simulink model "quadcopter_ex04_wind_test"  (R2025b)
settings: Solver=ode23t  StartTime=0.0  StopTime=timespot_spl(end)+2  FixedStep=0.01  MaxStep=1e-2  RelTol=1e-3  AbsTol=1e-3
PreLoadFcn:
  | [waypoints, timespot_spl, spline_data, spline_yaw, wayp_path_vis] = quadcopter_package_select_trajectory(2,true);
  | disp('Loaded path 2, round trip');
model workspace (MATLAB code in the model file):
  | load('xy_data_membrane.mat');
values from neighbouring files (symbols this model uses):
  wind_speed = 12    [quadcopter_ex04_wind_test_code.m]
undefined symbols (not defined in the file or in its folder): air_rho, battery_capacity, drone_leg, filtD_altitude, filtD_attitude, filtD_motor, filtD_position, filtD_yaw, filtM_altitude, filtM_attitude, filtM_position, filtM_yaw, filtSpd_motor, kd_altitude, kd_attitude, kd_motor, kd_position, kd_yaw, ki_altitude, ki_attitude, ki_motor, ki_position, ki_yaw, kp_altitude, kp_attitude, kp_motor, kp_position, kp_yaw, limit_altitude, limit_attitude, limit_motor, limit_yaw, pkgDensity, pkgSize, planedepth, pos2attitude, propeller, qc_motor, qd_area, qd_drag, spline_data, spline_yaw, timespot_spl, waypoints, X, Y, Z
libraries: sm_lib x77, nesl_utility x30, fl_lib x13, slpidlib x9, quadcopter_library x6, ee_lib x4, simulink x2, batteryecm_lib x1
(part 4 of 4)

== system quadcopter_ex04_wind_test/Quadcopter/Electrical/Control1 ==
  ref : Inport
  meas : Inport  Port=2
  Add : Sum  Inputs=+-
  Control : slpidlib/PID Controller  Controller=PID  Form=Parallel  TimeDomain=Continuous-time  UseExternalTs=off  SampleTime=-1  IntegratorMethod=Forward Euler  FilterMethod=Forward Euler  ControllerParametersSource=internal  P=kp  I=ki  UseKiTs=off  D=kd  UseExternalDerivativeSource=off  N=f_deriv  UseFilter=on  TunerSelectOption=Transfer Function Based (PID Tuner App)  ZeroCross=off  InitialConditionSource=internal  InitialConditionForIntegrator=0  InitialConditionForFilter=0  DifferentiatorICPrevScaledInput=0  ExternalReset=none  TrackingMode=off  Kt=1  LimitOutput=on  SatLimitsSource=internal  UpperSaturationLimit=max_trq_cmd  LowerSaturationLimit=-max_trq_cmd  LinearizeAsGain=on  AntiWindupMode=clamping  Kb=1  LimitIntegrator=off  UpperIntegratorSaturationLimit=inf  LowerIntegratorSaturationLimit=-inf  POutMin=[]  POutMax=[]  IOutMin=[]  IOutMax=[]  DOutMin=[]  DOutMax=[]  NOutMin=[]  NOutMax=[]  SumOutMin=[]  SumOutMax=[]  SaturationOutMin=[]  SaturationOutMax=[]  PParamMin=[]  PParamMax=[]  IParamMin=[]  IParamMax=[]  DParamMin=[]  DParamMax=[]  NParamMin=[]  NParamMax=[]  KbParamMin=[]  KbParamMax=[]  KtParamMin=[]  KtParamMax=[]  KbOutMin=[]  KbOutMax=[]  KtOutMin=[]  KtOutMax=[]  IntegratorOutMin=[]  IntegratorOutMax=[]  FilterOutMin=[]  FilterOutMax=[]  SumI1OutMin=[]  SumI1OutMax=[]  SumI2OutMin=[]  SumI2OutMax=[]  SumI3OutMin=[]  SumI3OutMax=[]  SumI4OutMin=[]  SumI4OutMax=[]  SumDOutMin=[]  SumDOutMax=[]  DifferentiatorOutMin=[]  DifferentiatorOutMax=[]  FilterDiffOutCoefMin=[]  FilterDiffOutCoefMax=[]  ReciprocalOutMin=[]  ReciprocalOutMax=[]  SumDenOutMin=[]  SumDenOutMax=[]  SumNumOutMin=[]  SumNumOutMax=[]  DivideOutMin=[]  DivideOutMax=[]  UdiffTsProdOutMin=[]  UdiffTsProdOutMax=[]  NTsProdOutMin=[]  NTsProdOutMax=[]  UintegralTsProdOutMin=[]  UintegralTsProdOutMax=[]  UngainTsProdOutMin=[]  UngainTsProdOutMax=[]  ClampingZeroOutDataTypeStr=Inherit: Inherit via back propagation  ClampingZeroOutMin=[]  ClampingZeroOutMax=[]  FilterDenConstantOutDataTypeStr=Inherit: Inherit via back propagation  FilterDenConstantOutMin=[]  FilterDenConstantOutMax=[]  PCopyOutDataTypeStr=Inherit: Inherit via back propagation  PCopyOutMin=[]  PCopyOutMax=[]  NCopyOutDataTypeStr=Inherit: Inherit via back propagation  NCopyOutMin=[]  NCopyOutMax=[]  IntegratorContinuousStateAttributes=''  IntegratorStateMustResolveToSignalObject=off  IntegratorRTWStateStorageClass=Auto  FilterContinuousStateAttributes=''  FilterStateMustResolveToSignalObject=off  FilterRTWStateStorageClass=Auto  ParallelPVariant=InternalParameters  IdealPVariant=Disabled  IVariant=InternalParameters  DVariant=InternalParameters  IntegratorVariant=Continuous  SatVariant=Enabled  AWVariant=ContClampingParallel  PCopyVariant=Disabled  TRVariant=Disabled  FdbkBlocksVariant=Forward  IdealPFdbkVariant=Disabled  SatFdbkVariant=Disabled  DerivativeFilterVariant=ContFilter  NVariant=InternalParameters  NCopyVariant=Disabled  FilterICVariant=InternalICsFilter  IntegratorICVariant=InternalICs  ExternalResetVariant=Disabled  TRSumVariant=Passthrough  SumFdbkVariant=Disabled  SumVariant=Sum_PID  TsampFilterVariant=InternalTs  TsampNgainVariant=Passthrough  TsampIntegralVariant=Disabled_SignalSpec  ExternalSaturationOutDataTypeStr=Inherit: Same as second input  DerivativeSourceVariant=ErrorSignal  PreIntVariant=InternalPreInt
  Mux : Mux  Inputs=2
  Scope : Scope  NumInputPorts=3
      settings: ActiveDisplayYMinimum=-575.93509  ActiveDisplayYMaximum=5183.41577  DataLoggingVariableName=ScopeData3
  Transfer Fcn1 : TransferFcn  Denominator=[f_spd 1]
  torque : Outport
  wires:
  Control/1 -> torque/1, Scope/3  "torque"
  meas/1 -> Transfer Fcn1/1  "Meas"
  ref/1 -> Add/1, Mux/1  "Ref"
  Add/1 -> Scope/2, Control/1  "error"
  Mux/1 -> Scope/1
  Transfer Fcn1/1 -> Add/2, Mux/2

== system quadcopter_ex04_wind_test/Quadcopter/Electrical/Control2 ==
  ref : Inport
  meas : Inport  Port=2
  Add : Sum  Inputs=+-
  Control : slpidlib/PID Controller  Controller=PID  Form=Parallel  TimeDomain=Continuous-time  UseExternalTs=off  SampleTime=-1  IntegratorMethod=Forward Euler  FilterMethod=Forward Euler  ControllerParametersSource=internal  P=kp  I=ki  UseKiTs=off  D=kd  UseExternalDerivativeSource=off  N=f_deriv  UseFilter=on  TunerSelectOption=Transfer Function Based (PID Tuner App)  ZeroCross=off  InitialConditionSource=internal  InitialConditionForIntegrator=0  InitialConditionForFilter=0  DifferentiatorICPrevScaledInput=0  ExternalReset=none  TrackingMode=off  Kt=1  LimitOutput=on  SatLimitsSource=internal  UpperSaturationLimit=max_trq_cmd  LowerSaturationLimit=-max_trq_cmd  LinearizeAsGain=on  AntiWindupMode=clamping  Kb=1  LimitIntegrator=off  UpperIntegratorSaturationLimit=inf  LowerIntegratorSaturationLimit=-inf  POutMin=[]  POutMax=[]  IOutMin=[]  IOutMax=[]  DOutMin=[]  DOutMax=[]  NOutMin=[]  NOutMax=[]  SumOutMin=[]  SumOutMax=[]  SaturationOutMin=[]  SaturationOutMax=[]  PParamMin=[]  PParamMax=[]  IParamMin=[]  IParamMax=[]  DParamMin=[]  DParamMax=[]  NParamMin=[]  NParamMax=[]  KbParamMin=[]  KbParamMax=[]  KtParamMin=[]  KtParamMax=[]  KbOutMin=[]  KbOutMax=[]  KtOutMin=[]  KtOutMax=[]  IntegratorOutMin=[]  IntegratorOutMax=[]  FilterOutMin=[]  FilterOutMax=[]  SumI1OutMin=[]  SumI1OutMax=[]  SumI2OutMin=[]  SumI2OutMax=[]  SumI3OutMin=[]  SumI3OutMax=[]  SumI4OutMin=[]  SumI4OutMax=[]  SumDOutMin=[]  SumDOutMax=[]  DifferentiatorOutMin=[]  DifferentiatorOutMax=[]  FilterDiffOutCoefMin=[]  FilterDiffOutCoefMax=[]  ReciprocalOutMin=[]  ReciprocalOutMax=[]  SumDenOutMin=[]  SumDenOutMax=[]  SumNumOutMin=[]  SumNumOutMax=[]  DivideOutMin=[]  DivideOutMax=[]  UdiffTsProdOutMin=[]  UdiffTsProdOutMax=[]  NTsProdOutMin=[]  NTsProdOutMax=[]  UintegralTsProdOutMin=[]  UintegralTsProdOutMax=[]  UngainTsProdOutMin=[]  UngainTsProdOutMax=[]  ClampingZeroOutDataTypeStr=Inherit: Inherit via back propagation  ClampingZeroOutMin=[]  ClampingZeroOutMax=[]  FilterDenConstantOutDataTypeStr=Inherit: Inherit via back propagation  FilterDenConstantOutMin=[]  FilterDenConstantOutMax=[]  PCopyOutDataTypeStr=Inherit: Inherit via back propagation  PCopyOutMin=[]  PCopyOutMax=[]  NCopyOutDataTypeStr=Inherit: Inherit via back propagation  NCopyOutMin=[]  NCopyOutMax=[]  IntegratorContinuousStateAttributes=''  IntegratorStateMustResolveToSignalObject=off  IntegratorRTWStateStorageClass=Auto  FilterContinuousStateAttributes=''  FilterStateMustResolveToSignalObject=off  FilterRTWStateStorageClass=Auto  ParallelPVariant=InternalParameters  IdealPVariant=Disabled  IVariant=InternalParameters  DVariant=InternalParameters  IntegratorVariant=Continuous  SatVariant=Enabled  AWVariant=ContClampingParallel  PCopyVariant=Disabled  TRVariant=Disabled  FdbkBlocksVariant=Forward  IdealPFdbkVariant=Disabled  SatFdbkVariant=Disabled  DerivativeFilterVariant=ContFilter  NVariant=InternalParameters  NCopyVariant=Disabled  FilterICVariant=InternalICsFilter  IntegratorICVariant=InternalICs  ExternalResetVariant=Disabled  TRSumVariant=Passthrough  SumFdbkVariant=Disabled  SumVariant=Sum_PID  TsampFilterVariant=InternalTs  TsampNgainVariant=Passthrough  TsampIntegralVariant=Disabled_SignalSpec  ExternalSaturationOutDataTypeStr=Inherit: Same as second input  DerivativeSourceVariant=ErrorSignal  PreIntVariant=InternalPreInt
  Mux : Mux  Inputs=2
  Scope : Scope  NumInputPorts=3
      settings: ActiveDisplayYMinimum=-51413.90485  ActiveDisplayYMaximum=107953.94315  DataLoggingVariableName=ScopeData3
  Transfer Fcn1 : TransferFcn  Denominator=[f_spd 1]
  torque : Outport
  wires:
  Control/1 -> torque/1, Scope/3  "torque"
  ref/1 -> Add/1, Mux/1
  Add/1 -> Scope/2, Control/1  "error"
  Mux/1 -> Scope/1
  meas/1 -> Transfer Fcn1/1
  Transfer Fcn1/1 -> Add/2, Mux/2

== system quadcopter_ex04_wind_test/Quadcopter/Electrical/Control3 ==
  ref : Inport
  meas : Inport  Port=2
  Add : Sum  Inputs=+-
  Control : slpidlib/PID Controller  Controller=PID  Form=Parallel  TimeDomain=Continuous-time  UseExternalTs=off  SampleTime=-1  IntegratorMethod=Forward Euler  FilterMethod=Forward Euler  ControllerParametersSource=internal  P=kp  I=ki  UseKiTs=off  D=kd  UseExternalDerivativeSource=off  N=f_deriv  UseFilter=on  TunerSelectOption=Transfer Function Based (PID Tuner App)  ZeroCross=off  InitialConditionSource=internal  InitialConditionForIntegrator=0  InitialConditionForFilter=0  DifferentiatorICPrevScaledInput=0  ExternalReset=none  TrackingMode=off  Kt=1  LimitOutput=on  SatLimitsSource=internal  UpperSaturationLimit=max_trq_cmd  LowerSaturationLimit=-max_trq_cmd  LinearizeAsGain=on  AntiWindupMode=clamping  Kb=1  LimitIntegrator=off  UpperIntegratorSaturationLimit=inf  LowerIntegratorSaturationLimit=-inf  POutMin=[]  POutMax=[]  IOutMin=[]  IOutMax=[]  DOutMin=[]  DOutMax=[]  NOutMin=[]  NOutMax=[]  SumOutMin=[]  SumOutMax=[]  SaturationOutMin=[]  SaturationOutMax=[]  PParamMin=[]  PParamMax=[]  IParamMin=[]  IParamMax=[]  DParamMin=[]  DParamMax=[]  NParamMin=[]  NParamMax=[]  KbParamMin=[]  KbParamMax=[]  KtParamMin=[]  KtParamMax=[]  KbOutMin=[]  KbOutMax=[]  KtOutMin=[]  KtOutMax=[]  IntegratorOutMin=[]  IntegratorOutMax=[]  FilterOutMin=[]  FilterOutMax=[]  SumI1OutMin=[]  SumI1OutMax=[]  SumI2OutMin=[]  SumI2OutMax=[]  SumI3OutMin=[]  SumI3OutMax=[]  SumI4OutMin=[]  SumI4OutMax=[]  SumDOutMin=[]  SumDOutMax=[]  DifferentiatorOutMin=[]  DifferentiatorOutMax=[]  FilterDiffOutCoefMin=[]  FilterDiffOutCoefMax=[]  ReciprocalOutMin=[]  ReciprocalOutMax=[]  SumDenOutMin=[]  SumDenOutMax=[]  SumNumOutMin=[]  SumNumOutMax=[]  DivideOutMin=[]  DivideOutMax=[]  UdiffTsProdOutMin=[]  UdiffTsProdOutMax=[]  NTsProdOutMin=[]  NTsProdOutMax=[]  UintegralTsProdOutMin=[]  UintegralTsProdOutMax=[]  UngainTsProdOutMin=[]  UngainTsProdOutMax=[]  ClampingZeroOutDataTypeStr=Inherit: Inherit via back propagation  ClampingZeroOutMin=[]  ClampingZeroOutMax=[]  FilterDenConstantOutDataTypeStr=Inherit: Inherit via back propagation  FilterDenConstantOutMin=[]  FilterDenConstantOutMax=[]  PCopyOutDataTypeStr=Inherit: Inherit via back propagation  PCopyOutMin=[]  PCopyOutMax=[]  NCopyOutDataTypeStr=Inherit: Inherit via back propagation  NCopyOutMin=[]  NCopyOutMax=[]  IntegratorContinuousStateAttributes=''  IntegratorStateMustResolveToSignalObject=off  IntegratorRTWStateStorageClass=Auto  FilterContinuousStateAttributes=''  FilterStateMustResolveToSignalObject=off  FilterRTWStateStorageClass=Auto  ParallelPVariant=InternalParameters  IdealPVariant=Disabled  IVariant=InternalParameters  DVariant=InternalParameters  IntegratorVariant=Continuous  SatVariant=Enabled  AWVariant=ContClampingParallel  PCopyVariant=Disabled  TRVariant=Disabled  FdbkBlocksVariant=Forward  IdealPFdbkVariant=Disabled  SatFdbkVariant=Disabled  DerivativeFilterVariant=ContFilter  NVariant=InternalParameters  NCopyVariant=Disabled  FilterICVariant=InternalICsFilter  IntegratorICVariant=InternalICs  ExternalResetVariant=Disabled  TRSumVariant=Passthrough  SumFdbkVariant=Disabled  SumVariant=Sum_PID  TsampFilterVariant=InternalTs  TsampNgainVariant=Passthrough  TsampIntegralVariant=Disabled_SignalSpec  ExternalSaturationOutDataTypeStr=Inherit: Same as second input  DerivativeSourceVariant=ErrorSignal  PreIntVariant=InternalPreInt
  Mux : Mux  Inputs=2
  Scope : Scope  NumInputPorts=3
      settings: ActiveDisplayYMinimum=-734.86159  ActiveDisplayYMaximum=6613.7543  DataLoggingVariableName=ScopeData3
  Transfer Fcn1 : TransferFcn  Denominator=[f_spd 1]
  torque : Outport
  wires:
  Control/1 -> torque/1, Scope/3  "torque"
  ref/1 -> Add/1, Mux/1
  Add/1 -> Scope/2, Control/1  "error"
  Mux/1 -> Scope/1
  meas/1 -> Transfer Fcn1/1
  Transfer Fcn1/1 -> Add/2, Mux/2

== system quadcopter_ex04_wind_test/Quadcopter/Electrical/Control4 ==
  ref : Inport
  meas : Inport  Port=2
  Add : Sum  Inputs=+-
  Control : slpidlib/PID Controller  Controller=PID  Form=Parallel  TimeDomain=Continuous-time  UseExternalTs=off  SampleTime=-1  IntegratorMethod=Forward Euler  FilterMethod=Forward Euler  ControllerParametersSource=internal  P=kp  I=ki  UseKiTs=off  D=kd  UseExternalDerivativeSource=off  N=f_deriv  UseFilter=on  TunerSelectOption=Transfer Function Based (PID Tuner App)  ZeroCross=off  InitialConditionSource=internal  InitialConditionForIntegrator=0  InitialConditionForFilter=0  DifferentiatorICPrevScaledInput=0  ExternalReset=none  TrackingMode=off  Kt=1  LimitOutput=on  SatLimitsSource=internal  UpperSaturationLimit=max_trq_cmd  LowerSaturationLimit=-max_trq_cmd  LinearizeAsGain=on  AntiWindupMode=clamping  Kb=1  LimitIntegrator=off  UpperIntegratorSaturationLimit=inf  LowerIntegratorSaturationLimit=-inf  POutMin=[]  POutMax=[]  IOutMin=[]  IOutMax=[]  DOutMin=[]  DOutMax=[]  NOutMin=[]  NOutMax=[]  SumOutMin=[]  SumOutMax=[]  SaturationOutMin=[]  SaturationOutMax=[]  PParamMin=[]  PParamMax=[]  IParamMin=[]  IParamMax=[]  DParamMin=[]  DParamMax=[]  NParamMin=[]  NParamMax=[]  KbParamMin=[]  KbParamMax=[]  KtParamMin=[]  KtParamMax=[]  KbOutMin=[]  KbOutMax=[]  KtOutMin=[]  KtOutMax=[]  IntegratorOutMin=[]  IntegratorOutMax=[]  FilterOutMin=[]  FilterOutMax=[]  SumI1OutMin=[]  SumI1OutMax=[]  SumI2OutMin=[]  SumI2OutMax=[]  SumI3OutMin=[]  SumI3OutMax=[]  SumI4OutMin=[]  SumI4OutMax=[]  SumDOutMin=[]  SumDOutMax=[]  DifferentiatorOutMin=[]  DifferentiatorOutMax=[]  FilterDiffOutCoefMin=[]  FilterDiffOutCoefMax=[]  ReciprocalOutMin=[]  ReciprocalOutMax=[]  SumDenOutMin=[]  SumDenOutMax=[]  SumNumOutMin=[]  SumNumOutMax=[]  DivideOutMin=[]  DivideOutMax=[]  UdiffTsProdOutMin=[]  UdiffTsProdOutMax=[]  NTsProdOutMin=[]  NTsProdOutMax=[]  UintegralTsProdOutMin=[]  UintegralTsProdOutMax=[]  UngainTsProdOutMin=[]  UngainTsProdOutMax=[]  ClampingZeroOutDataTypeStr=Inherit: Inherit via back propagation  ClampingZeroOutMin=[]  ClampingZeroOutMax=[]  FilterDenConstantOutDataTypeStr=Inherit: Inherit via back propagation  FilterDenConstantOutMin=[]  FilterDenConstantOutMax=[]  PCopyOutDataTypeStr=Inherit: Inherit via back propagation  PCopyOutMin=[]  PCopyOutMax=[]  NCopyOutDataTypeStr=Inherit: Inherit via back propagation  NCopyOutMin=[]  NCopyOutMax=[]  IntegratorContinuousStateAttributes=''  IntegratorStateMustResolveToSignalObject=off  IntegratorRTWStateStorageClass=Auto  FilterContinuousStateAttributes=''  FilterStateMustResolveToSignalObject=off  FilterRTWStateStorageClass=Auto  ParallelPVariant=InternalParameters  IdealPVariant=Disabled  IVariant=InternalParameters  DVariant=InternalParameters  IntegratorVariant=Continuous  SatVariant=Enabled  AWVariant=ContClampingParallel  PCopyVariant=Disabled  TRVariant=Disabled  FdbkBlocksVariant=Forward  IdealPFdbkVariant=Disabled  SatFdbkVariant=Disabled  DerivativeFilterVariant=ContFilter  NVariant=InternalParameters  NCopyVariant=Disabled  FilterICVariant=InternalICsFilter  IntegratorICVariant=InternalICs  ExternalResetVariant=Disabled  TRSumVariant=Passthrough  SumFdbkVariant=Disabled  SumVariant=Sum_PID  TsampFilterVariant=InternalTs  TsampNgainVariant=Passthrough  TsampIntegralVariant=Disabled_SignalSpec  ExternalSaturationOutDataTypeStr=Inherit: Same as second input  DerivativeSourceVariant=ErrorSignal  PreIntVariant=InternalPreInt
  Mux : Mux  Inputs=2
  Scope : Scope  NumInputPorts=3
      settings: ActiveDisplayYMinimum=3391.57745  ActiveDisplayYMaximum=7073.87438  DataLoggingVariableName=ScopeData3
  Transfer Fcn1 : TransferFcn  Denominator=[f_spd 1]
  torque : Outport
  wires:
  Control/1 -> torque/1, Scope/3  "torque"
  ref/1 -> Add/1, Mux/1
  Add/1 -> Scope/2, Control/1  "error"
  Mux/1 -> Scope/1
  meas/1 -> Transfer Fcn1/1
  Transfer Fcn1/1 -> Add/2, Mux/2

== system quadcopter_ex04_wind_test/Quadcopter/Electrical/Sensing Temperature ==
  PS-Simulink Converter : nesl_utility/PS-Simulink Converter  PhysicalDomain=network_engine_domain  SubClassName=ps_output  LeftPortType=input  RightPortType=output  PseudoPeriodic=off  Frequencies=[]  VectorFormat=1-D array  Unit=inherit  AffineConversion=off
  Temperature Sensor : fl_lib/Thermal/Thermal Sensors/Temperature Sensor  temperature_measure=foundation.enum.MeasurementReference.difference
  Thermal Reference : fl_lib/Thermal/Thermal Elements/Thermal Reference
  A : PMIOPort  Side=Left
  T : Outport
  wires:
  PS-Simulink Converter/1 -> T/1
  connections:
  Thermal Reference/LConn1 -- Temperature Sensor/RConn1
  Temperature Sensor/RConn2 -- PS-Simulink Converter/LConn1
  A/RConn1 -- Temperature Sensor/LConn1

== system quadcopter_ex04_wind_test/Quadcopter/Electrical/Sensor M1 ==
  Current Sensor : fl_lib/Electrical/Electrical Sensors/Current Sensor
  PS-Simulink Converter3 : nesl_utility/PS-Simulink Converter  PhysicalDomain=network_engine_domain  SubClassName=ps_output  LeftPortType=input  RightPortType=output  PseudoPeriodic=off  Frequencies=[]  VectorFormat=1-D array  Unit=inherit  AffineConversion=off
  + : PMIOPort  Side=Left
  - : PMIOPort  Port=2  Side=Right
  i : Outport
  wires:
  PS-Simulink Converter3/1 -> i/1
  connections:
  +/RConn1 -- Current Sensor/LConn1
  Current Sensor/RConn2 -- -/RConn1
  PS-Simulink Converter3/LConn1 -- Current Sensor/RConn1

== system quadcopter_ex04_wind_test/Quadcopter/Electrical/Sensor M2 ==
  Current Sensor : fl_lib/Electrical/Electrical Sensors/Current Sensor
  PS-Simulink Converter3 : nesl_utility/PS-Simulink Converter  PhysicalDomain=network_engine_domain  SubClassName=ps_output  LeftPortType=input  RightPortType=output  PseudoPeriodic=off  Frequencies=[]  VectorFormat=1-D array  Unit=inherit  AffineConversion=off
  + : PMIOPort  Side=Left
  - : PMIOPort  Port=2  Side=Right
  i : Outport
  wires:
  PS-Simulink Converter3/1 -> i/1
  connections:
  PS-Simulink Converter3/LConn1 -- Current Sensor/RConn1
  Current Sensor/RConn2 -- -/RConn1
  +/RConn1 -- Current Sensor/LConn1

== system quadcopter_ex04_wind_test/Quadcopter/Electrical/Sensor M3 ==
  Current Sensor : fl_lib/Electrical/Electrical Sensors/Current Sensor
  PS-Simulink Converter3 : nesl_utility/PS-Simulink Converter  PhysicalDomain=network_engine_domain  SubClassName=ps_output  LeftPortType=input  RightPortType=output  PseudoPeriodic=off  Frequencies=[]  VectorFormat=1-D array  Unit=inherit  AffineConversion=off
  + : PMIOPort  Side=Left
  - : PMIOPort  Port=2  Side=Right
  i : Outport
  wires:
  PS-Simulink Converter3/1 -> i/1
  connections:
  +/RConn1 -- Current Sensor/LConn1
  Current Sensor/RConn2 -- -/RConn1
  PS-Simulink Converter3/LConn1 -- Current Sensor/RConn1

== system quadcopter_ex04_wind_test/Quadcopter/Electrical/Sensor M4 ==
  Current Sensor : fl_lib/Electrical/Electrical Sensors/Current Sensor
  PS-Simulink Converter3 : nesl_utility/PS-Simulink Converter  PhysicalDomain=network_engine_domain  SubClassName=ps_output  LeftPortType=input  RightPortType=output  PseudoPeriodic=off  Frequencies=[]  VectorFormat=1-D array  Unit=inherit  AffineConversion=off
  + : PMIOPort  Side=Left
  - : PMIOPort  Port=2  Side=Right
  i : Outport
  wires:
  PS-Simulink Converter3/1 -> i/1
  connections:
  PS-Simulink Converter3/LConn1 -- Current Sensor/RConn1
  Current Sensor/RConn2 -- -/RConn1
  +/RConn1 -- Current Sensor/LConn1

== system quadcopter_ex04_wind_test/Quadcopter/Ground/Ground ==
  Ground : sm_lib/Body Elements/Brick Solid  BrickDimensions=[plane_x plane_y planedepth]  BrickDimensionsUnits=m  ExportEntireGeometry=off  InertiaType=CalculateFromGeometry  BasedOnType=Density  Density=1000  DensityUnits=kg/m^3  Mass=1  MassUnits=kg  CenterOfMass=[0 0 0]  CenterOfMassUnits=m  MomentsOfInertia=[1 1 1]  MomentsOfInertiaUnits=kg*m^2  ProductsOfInertia=[0 0 0]  ProductsOfInertiaUnits=kg*m^2  GraphicType=FromGeometry  MarkerShape=Sphere  MarkerSize=10  GraphicVisPropType=SimpleVisualProperties  GraphicDiffuseColor=[0.0 0.7 0.1]  GraphicOpacity=1  GraphicSpecularColor=[0.5 0.5 0.5 1.0]  GraphicAmbientColor=[0.15 0.15 0.15 1.0]  GraphicEmissiveColor=[0.0 0.0 0.0 1.0]  GraphicShininess=75  DoExposeReferenceFrame=on  SerializedFrames=<Frames><Frame><Id>Frame1</Id><Value><Name>Lp</Name><Origin><Source>GeometricFeature</Source><FeatureName>+z surface</FeatureName></Origin><PrimaryAxis><DefinedDirection>+Z</DefinedDirection><Source>ReferenceFrame</Source><SourceDirection>+Z</SourceDirection><FeatureName></FeatureName></PrimaryAxis><SecondaryAxis><DefinedDirection>+X</DefinedDirection><Source>ReferenceFrame</Source><SourceDirection>+X</SourceDirection><FeatureName></FeatureName></SecondaryAxis></Value></Frame></Frames>
  Transform Ground Center : sm_lib/Frames and Transforms/Rigid Transform  RotationMethod=None  FollAlignAxisA=+X  BaseAlignAxisA=+Y  FollAlignAxisB=+Y  BaseAlignAxisB=+Z  RotationStandardAxis=+Z  RotationAngle=0.0  RotationAngleUnits=deg  RotationArbitraryAxis=[0 0 1]  RotationSequenceAxes=FollowerAxes  RotationSequence=XYX  RotationSequenceAngles=[0 0 0]  RotationSequenceAnglesUnits=deg  RotationMatrix=[1 0 0; 0 1 0; 0 0 1]  Quaternion=[1 0 0 0]  TranslationMethod=Cartesian  TranslationCartesianOffset=[offset_x offset_y -planedepth/2]  TranslationCartesianOffsetUnits=m  TranslationStandardAxis=-Z  TranslationStandardOffset=0  TranslationStandardOffsetUnits=m  TranslationROffset=0  TranslationROffsetUnits=m  TranslationThetaOffset=0  TranslationThetaOffsetUnits=deg  TranslationZOffset=0  TranslationZOffsetUnits=m
  Lp : PMIOPort  Side=Right
  W : PMIOPort  Port=2  Side=Left
  connections:
  Lp/RConn1 -- Ground/LConn1
  Transform Ground Center/RConn1 -- Ground/RConn1
  W/RConn1 -- Transform Ground Center/LConn1

== system quadcopter_ex04_wind_test/Quadcopter/Ground/Trajectory ==
  Spline : sm_lib/Curves and Surfaces/Spline  DataPoints=wayp_path_vis  DataPointsUnits=m  EndConditionType=Natural  GraphicType=FromGeometry  MarkerShape=Sphere  MarkerSize=10  GraphicVisPropType=SimpleVisualProperties  GraphicDiffuseColor=[1.0 1.0 0.2]  GraphicOpacity=0.5  GraphicSpecularColor=[0.5 0.5 0.5 1.0]  GraphicAmbientColor=[0.15 0.15 0.15 1.0]  GraphicEmissiveColor=[0.0 0.0 0.0 1.0]  GraphicShininess=75
  Waypoints : sm_lib/Curves and Surfaces/Point Cloud  CoordinatesMatrix=unique(waypoints','rows')  CoordinatesMatrixUnits=m  GraphicType=MarkerCloud  GraphicSphereRadius=2e-1  GraphicSphereRadiusUnits=m  GraphicVisPropType=SimpleVisualProperties  GraphicDiffuseColor=[0.302 0.7451 0.9333]  GraphicOpacity=0.5  GraphicSpecularColor=[0.5 0.5 0.5 1.0]  GraphicAmbientColor=[0.15 0.15 0.15 1.0]  GraphicEmissiveColor=[0.0 0.0 0.0 1.0]  GraphicShininess=75
  W : PMIOPort  Side=Right
  connections:
  Spline/LConn1 -- W/RConn1 -- Waypoints/LConn1

== system quadcopter_ex04_wind_test/Quadcopter/Wind and Drag/Aerodynamic Drag ==
  vxRel : Inport
  vyRel : Inport  Port=2
  vzRel : Inport  Port=3
  nRoll : Inport  Port=4
  nPitch : Inport  Port=5
  nYaw : Inport  Port=6
  yaw : Inport  Port=7
  Body to World : Subsystem  mask{area_front=area_values.YZ, area_side=area_values.XZ, drag_front=drag_coeff.Cd_X, drag_side=drag_coeff.Cd_Y}
      mask prompts: area_front "Area Front (m^2)"; area_side "Area Side (m^2)"; drag_front "Drag Coefficient Front"; drag_side "Drag Coefficient Side"
  Mux4 : Mux  Inputs=3
  Mux5 : Mux  Inputs=3
  drag force X : Subsystem
  drag force Y : Subsystem
  drag force Z : Subsystem
  drag moment pitch : Subsystem
  drag moment roll : Subsystem
  drag moment yaw : Subsystem
  f : Outport
  t : Outport  Port=2
  wires:
  vxRel/1 -> drag force X/3(v)
  vyRel/1 -> drag force Y/3(v)
  vzRel/1 -> drag force Z/1(vz)
  nRoll/1 -> drag moment roll/1(v)
  nPitch/1 -> drag moment pitch/1(v)
  nYaw/1 -> drag moment yaw/1(v)
  drag force X/1(f) -> Mux4/1
  drag force Y/1(f) -> Mux4/2
  drag force Z/1(f) -> Mux4/3
  drag moment roll/1(f) -> Mux5/1
  drag moment pitch/1(f) -> Mux5/2
  drag moment yaw/1(f) -> Mux5/3
  Mux4/1 -> f/1
  Mux5/1 -> t/1
  yaw/1 -> Body to World/1(yaw)
  Body to World/1(areaX) -> drag force X/1(area)
  Body to World/3(areaY) -> drag force Y/1(area)
  Body to World/2(dragX) -> drag force X/2(Cd)
  Body to World/4(dragY) -> drag force Y/2(Cd)

== system quadcopter_ex04_wind_test/Quadcopter/6 DOF/R to X-Y-Z Extrinsic/Unwrap ==
  angle : Inport
  w : Inport  Port=2
  Fcn1 : Fcn  Expr=u(2) + (2*(u(1) > u(2)) - 1)*2*pi*floor(abs(u(1)-u(2))/(2*pi) + 0.5)
  Gain1 : Gain  SaturateOnIntegerOverflow=on  OutDataTypeStr=Inherit: Same as input  ParamDataTypeStr=Inherit: Same as input
  Gain3 : Gain  SaturateOnIntegerOverflow=on  OutDataTypeStr=Inherit: Same as input  ParamDataTypeStr=Inherit: Same as input
  Gain4 : Gain  SaturateOnIntegerOverflow=on  OutDataTypeStr=Inherit: Same as input  ParamDataTypeStr=Inherit: Same as input
  Integrator : Integrator  InitialConditionSource=external  AbsoluteTolerance=1e-3  ZeroCross=off
  Mux : Mux  Inputs=2
  unwrapped : Outport
  wires:
  Gain1/1 -> Mux/2, Integrator/2
  Gain3/1 -> Integrator/1
  Fcn1/1 -> Gain4/1
  Mux/1 -> Fcn1/1
  Integrator/1 -> Mux/1
  angle/1 -> Gain1/1
  Gain4/1 -> unwrapped/1
  w/1 -> Gain3/1

== system quadcopter_ex04_wind_test/Quadcopter/6 DOF/Roll Pitch/Calculate aPitch ==
  Roll Angle : Inport
  uvec : Inport  Port=2
  Asin : Trigonometry  Operator=asin
  Cos : Trigonometry  Operator=cos
  Divide : Product  Inputs=*/
  Divide1 : Product  Inputs=*/
  Selector : Selector  InputPortWidth=3  IndexOptions=Index vector (dialog)  Indices=[3]  OutputSizes=1
  magnitude : Fcn  Expr=sqrt(u(1)*u(1)+u(2)*u(2)+u(3)*u(3))
  Angle : Outport  VectorParamsAs1DForOutWhenUnconnected=off
  wires:
  Divide1/1 -> Asin/1
  uvec/1 -> magnitude/1, Selector/1
  magnitude/1 -> Divide1/2
  Selector/1 -> Divide/1
  Roll Angle/1 -> Cos/1
  Asin/1 -> Angle/1
  Divide/1 -> Divide1/1
  Cos/1 -> Divide/2

== system quadcopter_ex04_wind_test/Quadcopter/6 DOF/Roll Pitch/Calculate aRoll ==
  uvec : Inport
  Demux : Demux  Outputs=3
  Mux : Mux  Inputs=2
  Trigonometric Function1 : Trigonometry  Operator=atan2
  magnitude : Fcn  Expr=sqrt(u(1)*u(1)+u(2)*u(2))
  Angle : Outport  VectorParamsAs1DForOutWhenUnconnected=off
  wires:
  Demux/2 -> Mux/2
  magnitude/1 -> Trigonometric Function1/2
  Mux/1 -> magnitude/1
  Demux/3 -> Trigonometric Function1/1
  Trigonometric Function1/1 -> Angle/1
  uvec/1 -> Demux/1
  Demux/1 -> Mux/1

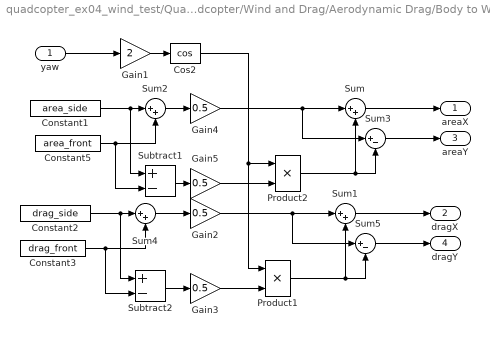
== system quadcopter_ex04_wind_test/Quadcopter/Wind and Drag/Aerodynamic Drag/Body to World ==
  yaw : Inport
  Constant1 : Constant  Value=area_side
  Constant2 : Constant  Value=drag_side
  Constant3 : Constant  Value=drag_front
  Constant5 : Constant  Value=area_front
  Cos2 : Trigonometry  Operator=cos
  Gain1 : Gain  Gain=2
  Gain{2..5} (4 alike) : Gain  Gain=0.5
  Product1 : Product
  Product2 : Product
  Subtract1 : Sum  Inputs=+-
  Subtract2 : Sum  Inputs=+-
  Sum{,1..2,4} (4 alike) : Sum  Inputs=|++
  Sum3 : Sum  Inputs=|+-
  Sum5 : Sum  Inputs=|+-
  areaX : Outport
  dragX : Outport  Port=2
  areaY : Outport  Port=3
  dragY : Outport  Port=4
  wires:
  Sum/1 -> areaX/1
  Sum3/1 -> areaY/1
  Gain5/1 -> Product2/2
  Gain4/1 -> Sum3/1, Sum/1
  Product2/1 -> Sum/2, Sum3/2
  Constant1/1 -> Subtract1/1, Sum2/1
  Constant5/1 -> Subtract1/2, Sum2/2
  Sum2/1 -> Gain4/1
  Subtract1/1 -> Gain5/1
  Gain1/1 -> Cos2/1
  yaw/1 -> Gain1/1
  Cos2/1 -> Product1/1, Product2/1
  Subtract2/1 -> Gain3/1
  Sum4/1 -> Gain2/1
  Constant3/1 -> Sum4/2, Subtract2/2
  Constant2/1 -> Sum4/1, Subtract2/1
  Product1/1 -> Sum5/2, Sum1/2
  Gain2/1 -> Sum1/1, Sum5/1
  Gain3/1 -> Product1/2
  Sum5/1 -> dragY/1
  Sum1/1 -> dragX/1

== system quadcopter_ex04_wind_test/Quadcopter/Wind and Drag/Aerodynamic Drag/drag force X ==
  area : Inport
  Cd : Inport  Port=2
  v : Inport  Port=3
  Constant : Constant  Value=rho_air/2
  Gain : Gain  Gain=-1
  Product : Product  Inputs=5
  Sign : Signum  ZeroCross=off
  Square : Math  Operator=square
  f : Outport
  wires:
  Square/1 -> Product/4
  Product/1 -> Gain/1
  Gain/1 -> f/1
  Constant/1 -> Product/1
  Cd/1 -> Product/3
  area/1 -> Product/2
  Sign/1 -> Product/5
  v/1 -> Sign/1, Square/1

== system quadcopter_ex04_wind_test/Quadcopter/Wind and Drag/Aerodynamic Drag/drag force Y ==
  area : Inport
  Cd : Inport  Port=2
  v : Inport  Port=3
  Constant : Constant  Value=rho_air/2
  Gain : Gain  Gain=-1
  Product : Product  Inputs=5
  Sign : Signum  ZeroCross=off
  Square : Math  Operator=square
  f : Outport
  wires:
  v/1 -> Sign/1, Square/1
  area/1 -> Product/2
  Sign/1 -> Product/5
  Gain/1 -> f/1
  Cd/1 -> Product/3
  Square/1 -> Product/4
  Product/1 -> Gain/1
  Constant/1 -> Product/1

== system quadcopter_ex04_wind_test/Quadcopter/Wind and Drag/Aerodynamic Drag/drag force Z ==
  vz : Inport
  Constant : Constant  Value=rho_air/2
  Constant1 : Constant  Value=area_values.XY
  Constant2 : Constant  Value=drag_coeff.Cd_Z
  Gain : Gain  Gain=-1
  Product : Product  Inputs=5
  Sign : Signum  ZeroCross=off
  Square : Math  Operator=square
  f : Outport
  wires:
  vz/1 -> Sign/1, Square/1
  Gain/1 -> f/1
  Square/1 -> Product/4
  Product/1 -> Gain/1
  Sign/1 -> Product/5
  Constant1/1 -> Product/2
  Constant/1 -> Product/1
  Constant2/1 -> Product/3

== system quadcopter_ex04_wind_test/Quadcopter/Wind and Drag/Aerodynamic Drag/drag moment pitch ==
  v : Inport
  Constant : Constant  Value=rho_air/2
  Constant1 : Constant  Value=area_values.Pitch
  Constant2 : Constant  Value=drag_coeff.Pitch
  Gain : Gain  Gain=-1
  Product : Product  Inputs=5
  Sign : Signum  ZeroCross=off
  Square : Math  Operator=square
  f : Outport
  wires:
  Product/1 -> Gain/1
  Constant2/1 -> Product/3
  v/1 -> Sign/1, Square/1
  Constant/1 -> Product/1
  Sign/1 -> Product/5
  Constant1/1 -> Product/2
  Gain/1 -> f/1
  Square/1 -> Product/4

== system quadcopter_ex04_wind_test/Quadcopter/Wind and Drag/Aerodynamic Drag/drag moment roll ==
  v : Inport
  Constant : Constant  Value=rho_air/2
  Constant1 : Constant  Value=area_values.Roll
  Constant2 : Constant  Value=drag_coeff.Roll
  Gain : Gain  Gain=-1
  Product : Product  Inputs=5
  Sign : Signum  ZeroCross=off
  Square : Math  Operator=square
  f : Outport
  wires:
  Product/1 -> Gain/1
  v/1 -> Sign/1, Square/1
  Constant/1 -> Product/1
  Constant1/1 -> Product/2
  Constant2/1 -> Product/3
  Square/1 -> Product/4
  Sign/1 -> Product/5
  Gain/1 -> f/1

== system quadcopter_ex04_wind_test/Quadcopter/Wind and Drag/Aerodynamic Drag/drag moment yaw ==
  v : Inport
  Constant : Constant  Value=rho_air/2
  Constant1 : Constant  Value=area_values.Yaw
  Constant2 : Constant  Value=drag_coeff.Yaw
  Gain : Gain  Gain=-1
  Product : Product  Inputs=5
  Sign : Signum  ZeroCross=off
  Square : Math  Operator=square
  f : Outport
  wires:
  Constant1/1 -> Product/2
  Sign/1 -> Product/5
  Constant/1 -> Product/1
  v/1 -> Sign/1, Square/1
  Gain/1 -> f/1
  Constant2/1 -> Product/3
  Square/1 -> Product/4
  Product/1 -> Gain/1

== matlab function quadcopter_ex04_wind_test/Maneuver Controller/Position Control/Calculate RBI ==
  data: R_BI output; attitude input
function R_BI  = Calculate_RBI(attitude)

phi   = attitude(1);
theta = attitude(2);
psi   = attitude(3);

% obtain the desired state
R_BI = [cos(theta)*cos(psi)                                    cos(theta)*sin(psi)                          -sin(theta);
    -cos(phi)*sin(psi)+sin(phi)*sin(theta)*cos(psi) cos(phi)*cos(psi)+sin(phi)*sin(theta)*sin(psi) sin(phi)*cos(theta);
    sin(phi)*sin(psi)+cos(phi)*sin(theta)*cos(psi) -sin(phi)*cos(psi)+cos(phi)*sin(theta)*sin(psi) cos(phi)*cos(theta)];

end
